simulink model "im_inv_model"  (R2026a)
settings: Solver=ode23tb  StopTime=param.sim.simlength  FixedStep=param.sim.tc  MaxStep=param.glb_time.tc  EnableMultiTasking=on
values from neighbouring files (symbols this model uses):
  param = struct()    [init_model.m]
undefined symbols (not defined in the file or in its folder): magnitude
libraries: fl_lib x53, nesl_utility x25, simulink x2, lithium_ion_battery x1, induction_machine x1, threephase_inductor_lib x1, dclink_with_center_tap x1, cstblocks_lti x1
(part 1 of 3)
settings Model: SimulationMode=accelerator  Creator=LTNBDA  LastModifiedBy=ltnbda
settings SolverCC: ZeroCrossControl=EnableAll
settings DataIOCC: MaxDataPoints=1  SignalLoggingSaveFormat=ModelDataLogs
settings OptimizationCC: InitFltsAndDblsToZero=on
settings DebuggingCC: SaveWithParameterizedLinksMsg=none  UnderspecifiedInitializationDetection=Classic  SignalResolutionControl=TryResolveAllWithWarning  MultiTaskDSMMsg=warning  MultiTaskCondExecSysMsg=none  MultiTaskRateTransMsg=warning
settings HardwareCC: ProdBitPerLong=64.0  ProdHWDeviceType=Generic->64-bit Embedded Processor (LP64)
settings SFSimCC: SimCustomHeaderCode=|
  | #include "mavgflt.h"
  | #include "mavgflt_simulink.h"
  | #include "bemf_obsv.h"
  | #include "bemf_obsv_simulink.h"
  | #include "bemf_obsv_load_est.h"
  | #include "bemf_obsv_load_est_simulink.h"
  | #include "dqvector_pi.h"
  | #include "dqvector_pi_simulink.h"
  | #include "sv_pwm_simulink.h"
  | #include "sv_pwm.h"
settings SFSimCC: SimUserSources=|
  | "mavgflt_simulink.c"
  | "mavgflt.c"
  | "bemf_obsv_simulink.c"
  | "bemf_obsv.c"
  | "bemf_obsv_load_est_simulink.c"
  | "bemf_obsv_load_est.c"
  | "dqvector_pi.c"
  | "dqvector_pi_simulink.c"
  | "sv_pwm_simulink.c"
  | "sv_pwm.c"
settings SFSimCC: SimUserIncludeDirs=|
  | include
  | src
settings GRTTargetCC: TargetFcnLib=ansi_tfl_tmw.mat  CombineOutputUpdateFcns=off  GRTInterface=on
settings SimscapeCC: SimscapeNormalizeSystem=off  SimscapeNominalValues="[{\"value\":\"1\",\"unit\":\"A\"},{\"value\":\"1\",\"unit\":\"bar\"},{\"value\":\"1\",\"unit\":\"cm^2\"},{\"value\":\"1\",\"unit\":\"cm^3/s\"},{\"value\":\"1\",\"unit\":\"kJ/kg\"},{\"value\":\"1\",\"unit\":\"kW\"},{\"value\":\"1\",\"unit\":\"l\"},{\"value\":\"1\",\"unit\":\"N\"},{\"value\":\"1\",\"unit\":\"N*m\"},{\"value\":\"1\",\"unit\":\"V\"}]"  SimscapeLogType=none  SimscapeLogDataHistory=5000.0

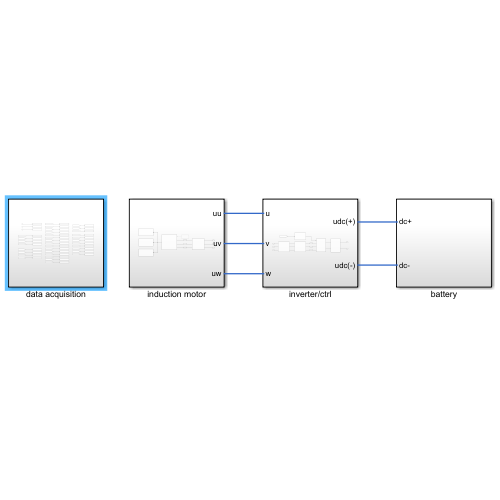
[thumbnail: Simulink's stored preview of the top-level diagram]
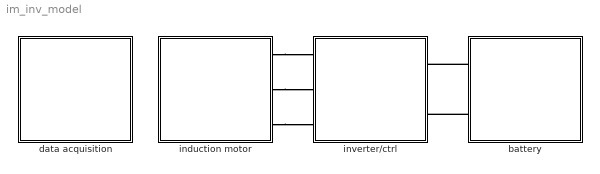
== system im_inv_model ==
  battery : Subsystem
  data acquisition : Subsystem
  induction motor : Subsystem
  inverter/ctrl : Subsystem
  connections:
  induction motor/RConn1 -- inverter/ctrl/LConn1
  induction motor/RConn2 -- inverter/ctrl/LConn2
  induction motor/RConn3 -- inverter/ctrl/LConn3
  battery/RConn1 -- inverter/ctrl/RConn1
  battery/RConn2 -- inverter/ctrl/RConn2

== system im_inv_model/battery ==
  To Workspace14 : ToWorkspace  VariableName=battery_data  SampleTime=param.glb_time.tc
      settings: MaxDataPoints=param.glb_time.Nc  Decimation=param.glb_time.decimation_tc
  lithium_ion_battery : lithium_ion_battery/lithium_ion_battery  Q=param.battery.pack_1.Q  number_of_cells=param.battery.pack_1.number_of_cells  E_1=param.battery.pack_1.E_1  E0=param.battery.pack_1.E0  E1=param.battery.pack_1.E1  E2=param.battery.pack_1.E2  E3=param.battery.pack_1.E3  Elog=param.battery.pack_1.Elog  R0=param.battery.pack_1.R0  R1=param.battery.pack_1.R1  C1=param.battery.pack_1.C1  M=param.battery.pack_1.M  alpha=param.battery.pack_1.alpha  soc_init=param.battery.pack_1.soc_init  ts_battery=param.glb_time.ts_dab  q1Kalman=param.battery.pack_1.q1Kalman  q2Kalman=param.battery.pack_1.q2Kalman  q3Kalman=param.battery.pack_1.q3Kalman  rKalman=param.battery.pack_1.rKalman  tc=param.glb_time.tc  enable_white_noise_m=0
  litium ion battery : Scope
      settings: ActiveDisplayYMinimum=-388.27149612119968  ActiveDisplayYMaximum=1221.0011073633038  DataLoggingVariableName=ScopeData3
  single_phase_ui_measure : Subsystem
  dc+ : PMIOPort  Side=Right
  dc- : PMIOPort  Port=2  Side=Right
  wires:
  lithium_ion_battery/1 -> To Workspace14/1, litium ion battery/1
  connections:
  lithium_ion_battery/RConn2 -- single_phase_ui_measure/LConn2
  single_phase_ui_measure/RConn1 -- dc+/RConn1
  lithium_ion_battery/RConn1 -- single_phase_ui_measure/LConn1
  dc-/RConn1 -- single_phase_ui_measure/RConn2

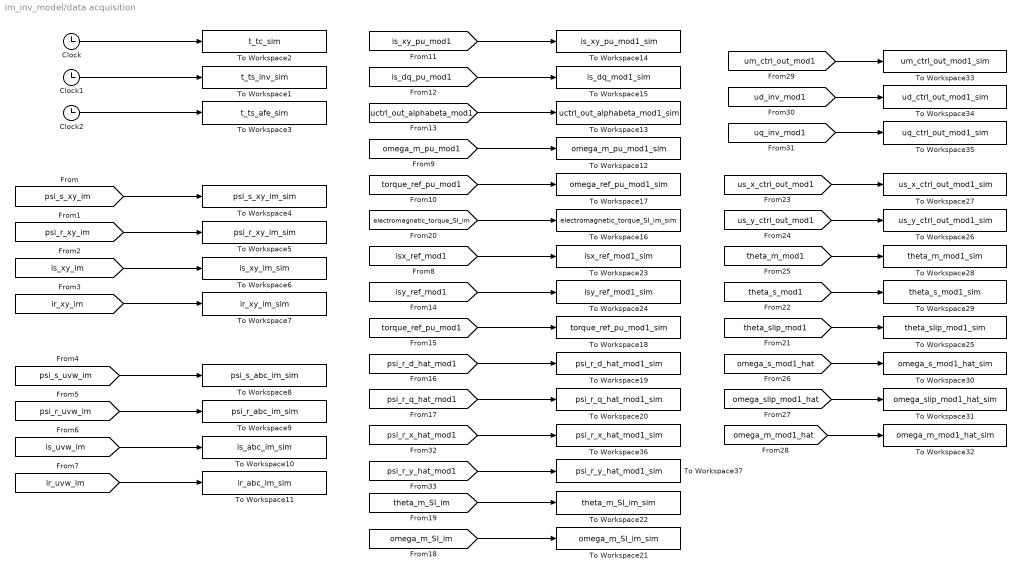
== system im_inv_model/data acquisition ==
  Clock : Clock
  Clock1 : Clock
  Clock2 : Clock
  To Workspace1 : ToWorkspace  VariableName=t_ts_inv_sim  SampleTime=param.glb_time.ts_inv
      settings: MaxDataPoints=param.glb_time.Ns_inv
  To Workspace10 : ToWorkspace  VariableName=is_abc_im_sim  SampleTime=param.glb_time.tc
      settings: MaxDataPoints=param.glb_time.Nc  Decimation=param.glb_time.decimation_tc
  To Workspace11 : ToWorkspace  VariableName=ir_abc_im_sim  SampleTime=param.glb_time.tc
      settings: MaxDataPoints=param.glb_time.Nc  Decimation=param.glb_time.decimation_tc
  To Workspace12 : ToWorkspace  VariableName=omega_m_pu_mod1_sim  SampleTime=param.glb_time.ts_inv
      settings: MaxDataPoints=param.glb_time.Ns_inv
  To Workspace13 : ToWorkspace  VariableName=uctrl_out_alphabeta_mod1_sim  SampleTime=param.glb_time.ts_inv
      settings: MaxDataPoints=param.glb_time.Ns_inv
  To Workspace14 : ToWorkspace  VariableName=is_xy_pu_mod1_sim  SampleTime=param.glb_time.ts_inv
      settings: MaxDataPoints=param.glb_time.Ns_inv
  To Workspace15 : ToWorkspace  VariableName=is_dq_mod1_sim  SampleTime=param.glb_time.ts_inv
      settings: MaxDataPoints=param.glb_time.Ns_inv
  To Workspace16 : ToWorkspace  VariableName=electromagnetic_torque_SI_im_sim  SampleTime=param.glb_time.ts_inv
      settings: MaxDataPoints=param.glb_time.Ns_inv
  To Workspace17 : ToWorkspace  VariableName=omega_ref_pu_mod1_sim  SampleTime=param.glb_time.ts_inv
      settings: MaxDataPoints=param.glb_time.Ns_inv
  To Workspace18 : ToWorkspace  VariableName=torque_ref_pu_mod1_sim  SampleTime=param.glb_time.ts_inv
      settings: MaxDataPoints=param.glb_time.Ns_inv
  To Workspace19 : ToWorkspace  VariableName=psi_r_d_hat_mod1_sim  SampleTime=param.glb_time.ts_inv
      settings: MaxDataPoints=param.glb_time.Ns_inv
  To Workspace2 : ToWorkspace  VariableName=t_tc_sim  SampleTime=param.glb_time.tc
      settings: MaxDataPoints=param.glb_time.Nc  Decimation=param.glb_time.decimation_tc
  To Workspace20 : ToWorkspace  VariableName=psi_r_q_hat_mod1_sim  SampleTime=param.glb_time.ts_inv
      settings: MaxDataPoints=param.glb_time.Ns_inv
  To Workspace21 : ToWorkspace  VariableName=omega_m_SI_im_sim  SampleTime=param.glb_time.ts_inv
      settings: MaxDataPoints=param.glb_time.Ns_inv
  To Workspace22 : ToWorkspace  VariableName=theta_m_SI_im_sim  SampleTime=param.glb_time.ts_inv
      settings: MaxDataPoints=param.glb_time.Ns_inv
  To Workspace23 : ToWorkspace  VariableName=isx_ref_mod1_sim  SampleTime=param.glb_time.ts_inv
      settings: MaxDataPoints=param.glb_time.Ns_inv
  To Workspace24 : ToWorkspace  VariableName=isy_ref_mod1_sim  SampleTime=param.glb_time.ts_inv
      settings: MaxDataPoints=param.glb_time.Ns_inv
  To Workspace25 : ToWorkspace  VariableName=theta_slip_mod1_sim  SampleTime=param.glb_time.ts_inv
      settings: MaxDataPoints=param.glb_time.Ns_inv
  To Workspace26 : ToWorkspace  VariableName=us_y_ctrl_out_mod1_sim  SampleTime=param.glb_time.ts_inv
      settings: MaxDataPoints=param.glb_time.Ns_inv
  To Workspace27 : ToWorkspace  VariableName=us_x_ctrl_out_mod1_sim  SampleTime=param.glb_time.ts_inv
      settings: MaxDataPoints=param.glb_time.Ns_inv
  To Workspace28 : ToWorkspace  VariableName=theta_m_mod1_sim  SampleTime=param.glb_time.ts_inv
      settings: MaxDataPoints=param.glb_time.Ns_inv
  To Workspace29 : ToWorkspace  VariableName=theta_s_mod1_sim  SampleTime=param.glb_time.ts_inv
      settings: MaxDataPoints=param.glb_time.Ns_inv
  To Workspace3 : ToWorkspace  VariableName=t_ts_afe_sim  SampleTime=param.glb_time.ts_inv
      settings: MaxDataPoints=param.glb_time.Ns_inv
  To Workspace30 : ToWorkspace  VariableName=omega_s_mod1_hat_sim  SampleTime=param.glb_time.ts_inv
      settings: MaxDataPoints=param.glb_time.Ns_inv
  To Workspace31 : ToWorkspace  VariableName=omega_slip_mod1_hat_sim  SampleTime=param.glb_time.ts_inv
      settings: MaxDataPoints=param.glb_time.Ns_inv
  To Workspace32 : ToWorkspace  VariableName=omega_m_mod1_hat_sim  SampleTime=param.glb_time.ts_inv
      settings: MaxDataPoints=param.glb_time.Ns_inv
  To Workspace33 : ToWorkspace  VariableName=um_ctrl_out_mod1_sim  SampleTime=param.glb_time.ts_inv
      settings: MaxDataPoints=param.glb_time.Ns_inv
  To Workspace34 : ToWorkspace  VariableName=ud_ctrl_out_mod1_sim  SampleTime=param.glb_time.ts_inv
      settings: MaxDataPoints=param.glb_time.Ns_inv
  To Workspace35 : ToWorkspace  VariableName=uq_ctrl_out_mod1_sim  SampleTime=param.glb_time.ts_inv
      settings: MaxDataPoints=param.glb_time.Ns_inv
  To Workspace36 : ToWorkspace  VariableName=psi_r_x_hat_mod1_sim  SampleTime=param.glb_time.ts_inv
      settings: MaxDataPoints=param.glb_time.Ns_inv
  To Workspace37 : ToWorkspace  VariableName=psi_r_y_hat_mod1_sim  SampleTime=param.glb_time.ts_inv
      settings: MaxDataPoints=param.glb_time.Ns_inv
  To Workspace4 : ToWorkspace  VariableName=psi_s_xy_im_sim  SampleTime=param.glb_time.tc
      settings: MaxDataPoints=param.glb_time.Nc  Decimation=param.glb_time.decimation_tc
  To Workspace5 : ToWorkspace  VariableName=psi_r_xy_im_sim  SampleTime=param.glb_time.tc
      settings: MaxDataPoints=param.glb_time.Nc  Decimation=param.glb_time.decimation_tc
  To Workspace6 : ToWorkspace  VariableName=is_xy_im_sim  SampleTime=param.glb_time.tc
      settings: MaxDataPoints=param.glb_time.Nc  Decimation=param.glb_time.decimation_tc
  To Workspace7 : ToWorkspace  VariableName=ir_xy_im_sim  SampleTime=param.glb_time.tc
      settings: MaxDataPoints=param.glb_time.Nc  Decimation=param.glb_time.decimation_tc
  To Workspace8 : ToWorkspace  VariableName=psi_s_abc_im_sim  SampleTime=param.glb_time.tc
      settings: MaxDataPoints=param.glb_time.Nc  Decimation=param.glb_time.decimation_tc
  To Workspace9 : ToWorkspace  VariableName=psi_r_abc_im_sim  SampleTime=param.glb_time.tc
      settings: MaxDataPoints=param.glb_time.Nc  Decimation=param.glb_time.decimation_tc
  wires:
  Clock/1 -> To Workspace2/1
  Clock1/1 -> To Workspace1/1
  Clock2/1 -> To Workspace3/1
  [psi_s_xy_im] -> To Workspace4/1
  [psi_r_xy_im] -> To Workspace5/1
  [is_xy_im] -> To Workspace6/1
  [ir_xy_im] -> To Workspace7/1
  [psi_s_uvw_im] -> To Workspace8/1
  [psi_r_uvw_im] -> To Workspace9/1
  [is_uvw_im] -> To Workspace10/1
  [ir_uvw_im] -> To Workspace11/1
  [is_dq_pu_mod1] -> To Workspace15/1
  [uctrl_out_alphabeta_mod1] -> To Workspace13/1
  [is_xy_pu_mod1] -> To Workspace14/1
  [omega_m_pu_mod1] -> To Workspace12/1
  [electromagnetic_torque_SI_im] -> To Workspace16/1
  [torque_ref_pu_mod1] -> To Workspace17/1
  [omega_m_SI_im] -> To Workspace21/1
  [torque_ref_pu_mod1] -> To Workspace18/1
  [psi_r_d_hat_mod1] -> To Workspace19/1
  [psi_r_q_hat_mod1] -> To Workspace20/1
  [theta_m_SI_im] -> To Workspace22/1
  [isx_ref_mod1] -> To Workspace23/1
  [isy_ref_mod1] -> To Workspace24/1
  [theta_slip_mod1] -> To Workspace25/1
  [us_x_ctrl_out_mod1] -> To Workspace27/1
  [us_y_ctrl_out_mod1] -> To Workspace26/1
  [theta_m_mod1] -> To Workspace28/1
  [theta_s_mod1] -> To Workspace29/1
  [omega_s_mod1_hat] -> To Workspace30/1
  [omega_slip_mod1_hat] -> To Workspace31/1
  [omega_m_mod1_hat] -> To Workspace32/1
  [um_ctrl_out_mod1] -> To Workspace33/1
  [ud_inv_mod1] -> To Workspace34/1
  [uq_inv_mod1] -> To Workspace35/1
  [psi_r_x_hat_mod1] -> To Workspace36/1
  [psi_r_y_hat_mod1] -> To Workspace37/1

== system im_inv_model/induction motor ==
  Inductor : fl_lib/Electrical/Electrical Elements/Inductor  l=1e-6 H  r=0 Ohm  g=1e-9 1/Ohm  i_specify=off  i_priority=None  i=0 A  i_nominal_specify=off  i_nominal_value=1  i_nominal_unit=A  v_specify=off  v_priority=None  v=0 V  v_nominal_specify=off  v_nominal_value=1  v_nominal_unit=V  i_L_specify=off  i_L_priority=High  i_L=0 A  i_L_nominal_specify=off  i_L_nominal_value=1  i_L_nominal_unit=A
  Inductor1 : fl_lib/Electrical/Electrical Elements/Inductor  l=1e-6 H  r=0 Ohm  g=1e-9 1/Ohm  i_specify=off  i_priority=None  i=0 A  i_nominal_specify=off  i_nominal_value=1  i_nominal_unit=A  v_specify=off  v_priority=None  v=0 V  v_nominal_specify=off  v_nominal_value=1  v_nominal_unit=V  i_L_specify=off  i_L_priority=High  i_L=0 A  i_L_nominal_specify=off  i_L_nominal_value=1  i_L_nominal_unit=A
  Inductor2 : fl_lib/Electrical/Electrical Elements/Inductor  l=1e-6 H  r=0 Ohm  g=1e-9 1/Ohm  i_specify=off  i_priority=None  i=0 A  i_nominal_specify=off  i_nominal_value=1  i_nominal_unit=A  v_specify=off  v_priority=None  v=0 V  v_nominal_specify=off  v_nominal_value=1  v_nominal_unit=V  i_L_specify=off  i_L_priority=High  i_L=0 A  i_L_nominal_specify=off  i_L_nominal_value=1  i_L_nominal_unit=A
  control performance evaluation : Subsystem
  induction motor : Subsystem
  load generator : Subsystem  Commented=on
  machine performance evaluation : Subsystem
  mechanical data : Subsystem
  threephase_vi_measures_stack : Subsystem
  uu : PMIOPort  Side=Right
  uv : PMIOPort  Port=2  Side=Right
  uw : PMIOPort  Port=3  Side=Right
  wires:
  induction motor/1(motor_data) -> control performance evaluation/1(machine_data), machine performance evaluation/1(machine_data), mechanical data/1(machine data)
  load generator/1(torque) -> induction motor/1(torque load)
  connections:
  induction motor/LConn2 -- Inductor1/LConn1
  threephase_vi_measures_stack/RConn1 -- Inductor/RConn1
  induction motor/LConn3 -- Inductor2/LConn1
  induction motor/LConn1 -- Inductor/LConn1
  threephase_vi_measures_stack/RConn2 -- Inductor1/RConn1
  threephase_vi_measures_stack/RConn3 -- Inductor2/RConn1
  threephase_vi_measures_stack/LConn1 -- uu/RConn1
  threephase_vi_measures_stack/LConn2 -- uv/RConn1
  threephase_vi_measures_stack/LConn3 -- uw/RConn1

== system im_inv_model/inverter//ctrl ==
  Inductor : fl_lib/Electrical/Electrical Elements/Inductor  l=1e-6 H  r=0 Ohm  g=1e-9 1/Ohm  i_specify=off  i_priority=None  i=0 A  i_nominal_specify=off  i_nominal_value=1  i_nominal_unit=A  v_specify=off  v_priority=None  v=0 V  v_nominal_specify=off  v_nominal_value=1  v_nominal_unit=V  i_L_specify=off  i_L_priority=High  i_L=0 A  i_L_nominal_specify=off  i_L_nominal_value=1  i_L_nominal_unit=A
  Inductor1 : fl_lib/Electrical/Electrical Elements/Inductor  l=1e-6 H  r=0 Ohm  g=1e-9 1/Ohm  i_specify=off  i_priority=None  i=0 A  i_nominal_specify=off  i_nominal_value=1  i_nominal_unit=A  v_specify=off  v_priority=None  v=0 V  v_nominal_specify=off  v_nominal_value=1  v_nominal_unit=V  i_L_specify=off  i_L_priority=High  i_L=0 A  i_L_nominal_specify=off  i_L_nominal_value=1  i_L_nominal_unit=A
  Inductor2 : fl_lib/Electrical/Electrical Elements/Inductor  l=1e-6 H  r=0 Ohm  g=1e-9 1/Ohm  i_specify=off  i_priority=None  i=0 A  i_nominal_specify=off  i_nominal_value=1  i_nominal_unit=A  v_specify=off  v_priority=None  v=0 V  v_nominal_specify=off  v_nominal_value=1  v_nominal_unit=V  i_L_specify=off  i_L_priority=High  i_L=0 A  i_L_nominal_specify=off  i_L_nominal_value=1  i_L_nominal_unit=A
  LFi : threephase_inductor_lib/threephase inductor  Lp=param.inv.hw.LFi H  L0=param.inv.hw.LFi_cm H  Rp=param.inv.hw.RLFi Ohm  R0=param.inv.hw.RLFi_cm Ohm  Lls=5e-6 H  uu_1_specify=off  uu_1_priority=None  uu_1=0 V  uu_1_nominal_specify=off  uu_1_nominal_value=1  uu_1_nominal_unit=V  uv_1_specify=off  uv_1_priority=None  uv_1=0 V  uv_1_nominal_specify=off  uv_1_nominal_value=1  uv_1_nominal_unit=V  uw_1_specify=off  uw_1_priority=None  uw_1=0 V  uw_1_nominal_specify=off  uw_1_nominal_value=1  uw_1_nominal_unit=V  uu_2_specify=off  uu_2_priority=None  uu_2=0 V  uu_2_nominal_specify=off  uu_2_nominal_value=1  uu_2_nominal_unit=V  uv_2_specify=off  uv_2_priority=None  uv_2=0 V  uv_2_nominal_specify=off  uv_2_nominal_value=1  uv_2_nominal_unit=V  uw_2_specify=off  uw_2_priority=None  uw_2=0 V  uw_2_nominal_specify=off  uw_2_nominal_value=1  uw_2_nominal_unit=V  iu_specify=off  iu_priority=None  iu=0 A  iu_nominal_specify=off  iu_nominal_value=1  iu_nominal_unit=A  iv_specify=off  iv_priority=None  iv=0 A  iv_nominal_specify=off  iv_nominal_value=1  iv_nominal_unit=A  iw_specify=off  iw_priority=None  iw=0 A  iw_nominal_specify=off  iw_nominal_value=1  iw_nominal_unit=A
  dc_source : Subsystem
  im_ctrl : Subsystem
  inverter : Subsystem
  threephase_vi_measures_stack : Subsystem
  u : PMIOPort  Side=Left
  v : PMIOPort  Port=2  Side=Left
  w : PMIOPort  Port=3  Side=Left
  udc(+) : PMIOPort  Port=4  Side=Right
  udc(-) : PMIOPort  Port=5  Side=Right
  wires:
  [theta_m_mod1] -> im_ctrl/1(theta_m)
  im_ctrl/1(u_ctrl_alphabeta) -> inverter/1(uab)
  connections:
  LFi/RConn1 -- Inductor/LConn1
  Inductor1/LConn1 -- LFi/RConn2
  LFi/RConn3 -- Inductor2/LConn1
  threephase_vi_measures_stack/LConn1 -- LFi/LConn1
  threephase_vi_measures_stack/LConn2 -- LFi/LConn2
  threephase_vi_measures_stack/LConn3 -- LFi/LConn3
  threephase_vi_measures_stack/RConn3 -- w/RConn1
  threephase_vi_measures_stack/RConn2 -- v/RConn1
  threephase_vi_measures_stack/RConn1 -- u/RConn1
  inverter/LConn1 -- Inductor/RConn1
  inverter/LConn2 -- Inductor1/RConn1
  inverter/LConn3 -- Inductor2/RConn1
  dc_source/RConn1 -- inverter/RConn1
  dc_source/RConn2 -- inverter/RConn2
  dc_source/LConn1 -- udc(+)/RConn1
  dc_source/LConn2 -- udc(-)/RConn1

== system im_inv_model/battery/single_phase_ui_measure ==
  Bus Creator : BusCreator  Inputs=2
  Current Sensor : fl_lib/Electrical/Electrical Sensors/Current Sensor
  Selector : Selector  InputPortWidth=2  IndexOptions=Index vector (dialog)  Indices=2  OutputSizes=1
  Selector1 : Selector  InputPortWidth=2  IndexOptions=Index vector (dialog)  Indices=1  OutputSizes=1
  Voltage Sensor : fl_lib/Electrical/Electrical Sensors/Voltage Sensor
  dab input modA : Scope  NumInputPorts=2
      settings: ActiveDisplayYMinimum=-2114.9540849373507  ActiveDisplayYMaximum=18648.004171529876  DataLoggingVariableName=ScopeData2
  iph : nesl_utility/PS-Simulink Converter  PhysicalDomain=network_engine_domain  SubClassName=ps_output  LeftPortType=input  RightPortType=output  PseudoPeriodic=off  Frequencies=[]  VectorFormat=1-D array  Unit=A  AffineConversion=off
  uph : nesl_utility/PS-Simulink Converter  PhysicalDomain=network_engine_domain  SubClassName=ps_output  LeftPortType=input  RightPortType=output  PseudoPeriodic=off  Frequencies=[]  VectorFormat=1-D array  Unit=V  AffineConversion=off
  Udc(+) : PMIOPort  Side=Left
  udc(+) : PMIOPort  Port=2  Side=Right
  Udc(-) : PMIOPort  Port=3  Side=Left
  udc(-) : PMIOPort  Port=4  Side=Right
  tag scope: current_battery=global, voltage_battery=global
  wires:
  Bus Creator/1 -> Selector/1, Selector1/1  "ui_data"
  iph/1 -> Bus Creator/1  "iph"
  uph/1 -> Bus Creator/2  "uph"
  Selector1/1 -> [current_battery], dab input modA/1  "current_battery"
  Selector/1 -> dab input modA/2, [voltage_battery]  "voltage_battery"
  connections:
  iph/LConn1 -- Current Sensor/RConn1
  Voltage Sensor/LConn1 -- Current Sensor/LConn1 -- Udc(+)/RConn1
  Current Sensor/RConn2 -- udc(+)/RConn1
  Voltage Sensor/RConn1 -- uph/LConn1
  Voltage Sensor/RConn2 -- Udc(-)/RConn1 -- udc(-)/RConn1

== system im_inv_model/induction motor/control performance evaluation ==
  machine_data : Inport
  adc2dq_s_1 : Subsystem
  adc2dq_s_2 : Subsystem
  adc2dq_slip_1 : Subsystem
  adc2dq_slip_2 : Subsystem
  ir_uvw : BusSelector  OutputSignals=iru(A),irv(A),irw(A)  OutputAsBus=on
  is_uvw : BusSelector  OutputSignals=isu(A),isv(A),isw(A)  OutputAsBus=on
  psi_r_uvw : BusSelector  OutputSignals=psi_r_u(Vs),psi_r_v(Vs),psi_r_w(Vs)  OutputAsBus=on
  psi_s_uvw : BusSelector  OutputSignals=psi_s_u(Vs),psi_s_v(Vs),psi_s_w(Vs)  OutputAsBus=on
  stator/rotor uvw currents : Scope  NumInputPorts=2
      settings: ActiveDisplayYMinimum=-767.52442584692187  ActiveDisplayYMaximum=813.0675363801156  DataLoggingVariableName=ScopeData15
  stator/rotor uvw fluxes : Scope  NumInputPorts=2
      settings: ActiveDisplayYMinimum=-1.236467692960036  ActiveDisplayYMaximum=1.3517472693614645  DataLoggingVariableName=ScopeData16
  stator/rotor xy currents : Scope  NumInputPorts=2
      settings: ActiveDisplayYMinimum=-2297.8110392737149  ActiveDisplayYMaximum=257.87338844640192
  stator/rotor xy fluxes : Scope  NumInputPorts=2
      settings: ActiveDisplayYMinimum=-2.073456127351001  ActiveDisplayYMaximum=0.70751576648044434  DataLoggingVariableName=ScopeData2
  tag scope: ir_uvw_im=global, is_uvw_im=global, psi_r_uvw_im=global, psi_s_uvw_im=global
  wires:
  machine_data/1 -> psi_s_uvw/1, psi_r_uvw/1, is_uvw/1, ir_uvw/1
  psi_s_uvw/1 -> [psi_s_uvw_im], adc2dq_s_1/1(abc)
  adc2dq_s_1/1(dq) -> stator/rotor xy fluxes/1  "psi_s_xy"
  psi_r_uvw/1 -> [psi_r_uvw_im], adc2dq_slip_1/1(abc)
  adc2dq_slip_1/1(dq) -> stator/rotor xy fluxes/2  "psi_r_xy"
  adc2dq_slip_2/1(dq) -> stator/rotor xy currents/2  "ir_xy"
  adc2dq_s_2/1(dq) -> stator/rotor xy currents/1  "is_xy"
  is_uvw/1 -> [is_uvw_im], adc2dq_s_2/1(abc)
  ir_uvw/1 -> [ir_uvw_im], adc2dq_slip_2/1(abc)
  [is_uvw_im] -> stator/rotor uvw currents/1
  [ir_uvw_im] -> stator/rotor uvw currents/2
  [psi_r_uvw_im] -> stator/rotor uvw fluxes/2
  [psi_s_uvw_im] -> stator/rotor uvw fluxes/1

== system im_inv_model/induction motor/induction motor ==
  torque load : Inport
  Gain : Gain  Gain=-1
  Ideal Rotational Motion Sensor : fl_lib/Mechanical/Mechanical Sensors/Ideal Rotational Motion Sensor  reference=foundation.enum.MeasurementReference.difference  acceleration_port=false  velocity_port=true  position_port=true  wrap_angle=false  offset=0 rad
  Ideal Torque Source : fl_lib/Mechanical/Mechanical Sources/Ideal Torque Source
  Mechanical Rotational Reference : fl_lib/Mechanical/Rotational Elements/Mechanical Rotational Reference
  Mechanical Rotational Reference1 : fl_lib/Mechanical/Rotational Elements/Mechanical Rotational Reference
  Open Circuit : fl_lib/Electrical/Electrical Elements/Open Circuit  v_specify=off  v_priority=None  v=0 V  v_nominal_specify=off  v_nominal_value=1  v_nominal_unit=V
  PS Gain : fl_lib/Physical Signals/Functions/PS Gain  gain=-1
  PS Transfer Function : fl_lib/Physical Signals/Linear Operators/PS Transfer Function  transfer_function_type=foundation.enum.transfer_function_type.lag  T=1/50 s  T1=2 s  T2=1 s  reset_method=foundation.enum.IntegratorResetSpec.None  initial_condition_spec=foundation.enum.IntegratorICSpec.Internal  y0=0 N*m
  PS-Simulink Converter24 : nesl_utility/PS-Simulink Converter  PhysicalDomain=network_engine_domain  SubClassName=ps_output  LeftPortType=input  RightPortType=output  PseudoPeriodic=off  Frequencies=[]  VectorFormat=1-D array  Unit=rad  AffineConversion=off
  Simulink-PS Converter : nesl_utility/Simulink-PS Converter  PhysicalDomain=network_engine_domain  SubClassName=ps_input  LeftPortType=input  RightPortType=output  PseudoPeriodic=off  Frequencies=[]  NoiseDistribution=none  NoiseParameters=[]  Unit=N*m  AffineConversion=off  FilteringAndDerivatives=provide  SimscapeFilterOrder=1  InputFilterTimeConstant=0.001  UdotUserProvided=0
  poliphase_induction_machine1 : induction_machine/poliphase_induction_machine  Rs_m=param.im.machine.Rs  Ls_m=param.im.machine.Ls  Lm_m=param.im.machine.Lm  Lr_m=param.im.machine.Lr  Rr_m=param.im.machine.Rr  Jm_m=param.im.machine.Jm  bm_m=param.im.machine.load_friction  cp_m=param.im.machine.pp
  uu : PMIOPort  Side=Left
  uv : PMIOPort  Port=2  Side=Left
  uw : PMIOPort  Port=3  Side=Left
  motor_data : Outport
  tag scope: rotor_phase_m_encoder=global
  wires:
  torque load/1 -> Simulink-PS Converter/1
  PS-Simulink Converter24/1 -> Gain/1
  Gain/1 -> [rotor_phase_m_encoder]
  poliphase_induction_machine1/1 -> motor_data/1
  connections:
  Ideal Torque Source/LConn1 -- poliphase_induction_machine1/RConn1 -- Ideal Rotational Motion Sensor/RConn1
  Mechanical Rotational Reference/LConn1 -- Ideal Torque Source/RConn2
  PS Transfer Function/RConn1 -- PS Gain/LConn1
  Simulink-PS Converter/RConn1 -- PS Transfer Function/LConn1
  PS Gain/RConn1 -- Ideal Torque Source/RConn1
  Mechanical Rotational Reference1/LConn1 -- Ideal Rotational Motion Sensor/LConn1
  Ideal Rotational Motion Sensor/RConn3 -- PS-Simulink Converter24/LConn1
  poliphase_induction_machine1/LConn1 -- uu/RConn1
  poliphase_induction_machine1/LConn2 -- uv/RConn1
  poliphase_induction_machine1/LConn3 -- uw/RConn1
  Open Circuit/LConn1 -- poliphase_induction_machine1/LConn4

== system im_inv_model/induction motor/load generator ==
  Gain3 : Gain
  RampSlow : simulink/Sources/Ramp  slope=param.im.load.Tload/param.im.load.timeRamp/param.sim.simlength*2  start=param.im.load.start_load_ramp  InitialOutput=0
  Saturation : Saturate  UpperLimit=param.im.load.Tload  LowerLimit=-param.im.load.Tload
  Step : Step  FinalValue=param.im.load.Tload  SampleTime=0
  torque : Outport
  wires:
  Gain3/1 -> torque/1
  RampSlow/1 -> Saturation/1
  Step/1 -> Gain3/1

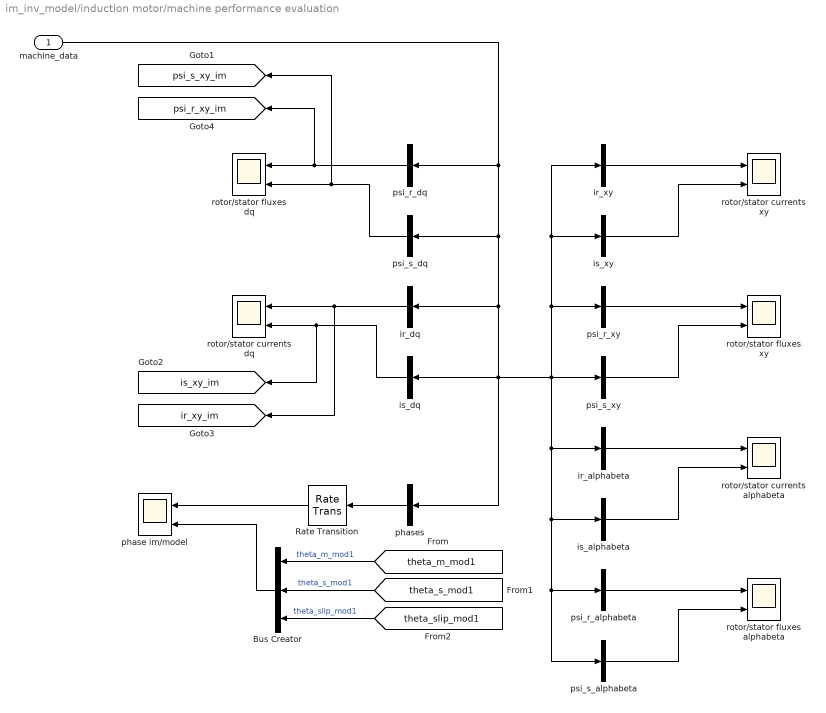
== system im_inv_model/induction motor/machine performance evaluation ==
  machine_data : Inport
  Bus Creator : BusCreator  Inputs=3
  Rate Transition : RateTransition
  ir_alphabeta : BusSelector  OutputSignals=ir_alpha(A),ir_beta(A)  OutputAsBus=on
  ir_dq : BusSelector  OutputSignals=ird(A),irq(A)  OutputAsBus=on
  ir_xy : BusSelector  OutputSignals=irx(A),iry(A)  OutputAsBus=on
  is_alphabeta : BusSelector  OutputSignals=is_alpha(A),is_beta(A)  OutputAsBus=on
  is_dq : BusSelector  OutputSignals="isd  (A),isq(A)"  OutputAsBus=on
  is_xy : BusSelector  OutputSignals=isx(A),isy(A)  OutputAsBus=on
  phase im/model : Scope  NumInputPorts=2
      settings: ActiveDisplayYMinimum=-3.9265862737533843  ActiveDisplayYMaximum=3.9260094563988228  DataLoggingVariableName=ScopeData17
  phases : BusSelector  OutputSignals=rotor_phase_electrical(rad),stator_phase_electrical(rad),slip_phase_electrical(rad)  OutputAsBus=on
  psi_r_alphabeta : BusSelector  OutputSignals=psi_r_alpha(Vs),psi_r_beta(Vs)  OutputAsBus=on
  psi_r_dq : BusSelector  OutputSignals=psi_r_d(Vs),psi_r_q(Vs)  OutputAsBus=on
  psi_r_xy : BusSelector  OutputSignals=psi_r_x(Vs),psi_r_y(Vs)  OutputAsBus=on
  psi_s_alphabeta : BusSelector  OutputSignals=psi_s_alpha(Vs),psi_s_beta(Vs)  OutputAsBus=on
  psi_s_dq : BusSelector  OutputSignals=psi_s_d(Vs),psi_s_q(Vs)  OutputAsBus=on
  psi_s_xy : BusSelector  OutputSignals=psi_s_x(Vs),psi_s_y(Vs)  OutputAsBus=on
  rotor/stator currents alphabeta : Scope  NumInputPorts=2
      settings: ActiveDisplayYMinimum=-755.39541757603456  ActiveDisplayYMaximum=755.78854721223524  DataLoggingVariableName=ScopeData13
  rotor/stator currents dq : Scope  NumInputPorts=2
      settings: ActiveDisplayYMinimum=-890.18338057152221  ActiveDisplayYMaximum=1029.0815378849704  DataLoggingVariableName=ScopeData3
  rotor/stator currents xy : Scope  NumInputPorts=2
      settings: ActiveDisplayYMinimum=-752.721270314659  ActiveDisplayYMaximum=755.87183047398014  DataLoggingVariableName=ScopeData6
  rotor/stator fluxes alphabeta : Scope  NumInputPorts=2
      settings: ActiveDisplayYMinimum=-2.3042822009960924  ActiveDisplayYMaximum=2.3048133761652672  DataLoggingVariableName=ScopeData14
  rotor/stator fluxes dq : Scope  NumInputPorts=2
      settings: ActiveDisplayYMinimum=-1.3704704510731207  ActiveDisplayYMaximum=1.3704905297766097
  rotor/stator fluxes xy : Scope  NumInputPorts=2
      settings: ActiveDisplayYMinimum=-1.4064321862490787  ActiveDisplayYMaximum=1.4064895725533888  DataLoggingVariableName=ScopeData12
  tag scope: ir_xy_im=global, is_xy_im=global, psi_r_xy_im=global, psi_s_xy_im=global
  wires:
  psi_r_dq/1 -> [psi_r_xy_im], rotor/stator fluxes dq/1
  psi_s_dq/1 -> [psi_s_xy_im], rotor/stator fluxes dq/2
  ir_dq/1 -> [ir_xy_im], rotor/stator currents dq/1
  is_dq/1 -> [is_xy_im], rotor/stator currents dq/2
  is_xy/1 -> rotor/stator currents xy/2
  ir_xy/1 -> rotor/stator currents xy/1
  psi_r_xy/1 -> rotor/stator fluxes xy/1
  psi_s_xy/1 -> rotor/stator fluxes xy/2
  psi_s_alphabeta/1 -> rotor/stator fluxes alphabeta/2
  psi_r_alphabeta/1 -> rotor/stator fluxes alphabeta/1
  machine_data/1 -> psi_r_dq/1, ir_dq/1, phases/1, psi_s_alphabeta/1, psi_r_alphabeta/1, is_alphabeta/1, ir_alphabeta/1, psi_s_xy/1, ir_xy/1, is_xy/1, psi_r_xy/1, is_dq/1, psi_s_dq/1
  ir_alphabeta/1 -> rotor/stator currents alphabeta/1
  is_alphabeta/1 -> rotor/stator currents alphabeta/2
  phases/1 -> Rate Transition/1
  [theta_m_mod1] -> Bus Creator/1  "theta_m_mod1"
  [theta_slip_mod1] -> Bus Creator/3  "theta_slip_mod1"
  Bus Creator/1 -> phase im/model/2
  [theta_s_mod1] -> Bus Creator/2  "theta_s_mod1"
  Rate Transition/1 -> phase im/model/1

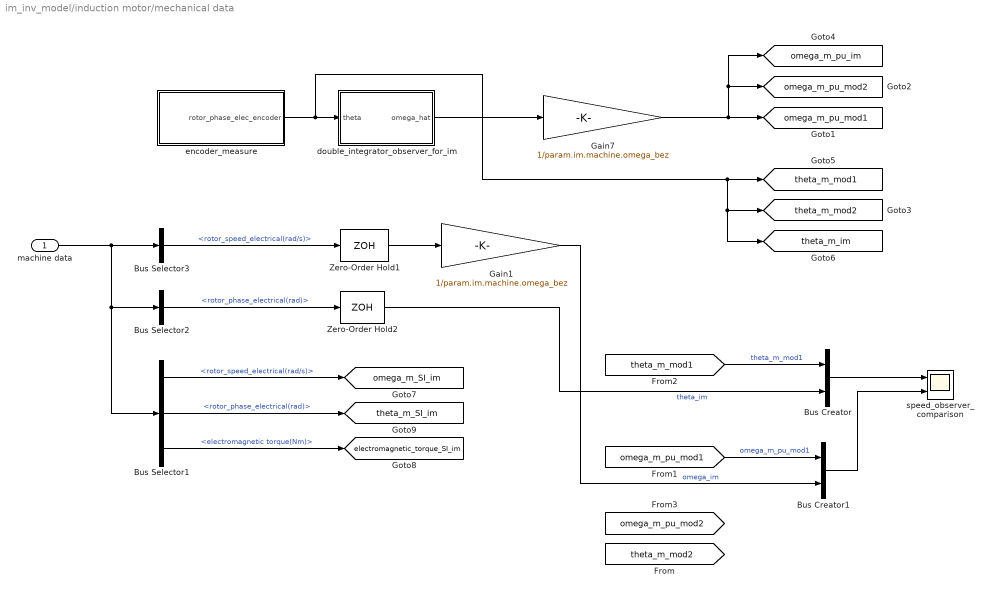
== system im_inv_model/induction motor/mechanical data ==
  machine data : Inport
  Bus Creator : BusCreator  Inputs=2
  Bus Creator1 : BusCreator  Inputs=2
  Bus Selector1 : BusSelector  OutputSignals=rotor_speed_electrical(rad/s),rotor_phase_electrical(rad),electromagnetic torque(Nm)
  Bus Selector2 : BusSelector  OutputSignals=rotor_phase_electrical(rad)
  Bus Selector3 : BusSelector  OutputSignals=rotor_speed_electrical(rad/s)
  Gain1 : Gain  Gain=1/param.im.machine.omega_bez
  Gain7 : Gain  Gain=1/param.im.machine.omega_bez
  Zero-Order Hold1 : ZeroOrderHold  SampleTime=param.glb_time.ts_inv
  Zero-Order Hold2 : ZeroOrderHold  SampleTime=param.glb_time.ts_inv
  double_integrator_observer_for_im : Subsystem
  encoder_measure : Subsystem
  speed_observer_comparison : Scope  NumInputPorts=2
      settings: ActiveDisplayYMinimum=-0.069232829506416654  ActiveDisplayYMaximum=0.62309538771470585  DataLoggingVariableName=ScopeData8
  tag scope: electromagnetic_torque_SI_im=global, omega_m_SI_im=global, omega_m_pu_im=global, omega_m_pu_mod1=global, omega_m_pu_mod2=global, theta_m_SI_im=global, theta_m_im=global, theta_m_mod1=global, theta_m_mod2=global
  wires:
  encoder_measure/1(rotor_phase_elec_encoder) -> [theta_m_mod1], [theta_m_im], [theta_m_mod2], double_integrator_observer_for_im/1(theta)
  machine data/1 -> Bus Selector1/1, Bus Selector2/1, Bus Selector3/1
  Bus Selector3/1 -> Zero-Order Hold1/1  "<rotor_speed_electrical(rad/s)>"
  Bus Selector2/1 -> Zero-Order Hold2/1  "<rotor_phase_electrical(rad)>"
  Gain7/1 -> [omega_m_pu_mod1], [omega_m_pu_mod2], [omega_m_pu_im]
  Bus Selector1/1 -> [omega_m_SI_im]  "<rotor_speed_electrical(rad/s)>"
  Bus Selector1/3 -> [electromagnetic_torque_SI_im]  "<electromagnetic torque(Nm)>"
  Bus Selector1/2 -> [theta_m_SI_im]  "<rotor_phase_electrical(rad)>"
  double_integrator_observer_for_im/1(omega_hat) -> Gain7/1
  [theta_m_mod1] -> Bus Creator/1  "theta_m_mod1"
  [omega_m_pu_mod1] -> Bus Creator1/1  "omega_m_pu_mod1"
  Bus Creator/1 -> speed_observer_comparison/1
  Bus Creator1/1 -> speed_observer_comparison/2
  Zero-Order Hold2/1 -> Bus Creator/2  "theta_im"
  Zero-Order Hold1/1 -> Gain1/1
  Gain1/1 -> Bus Creator1/2  "omega_im"

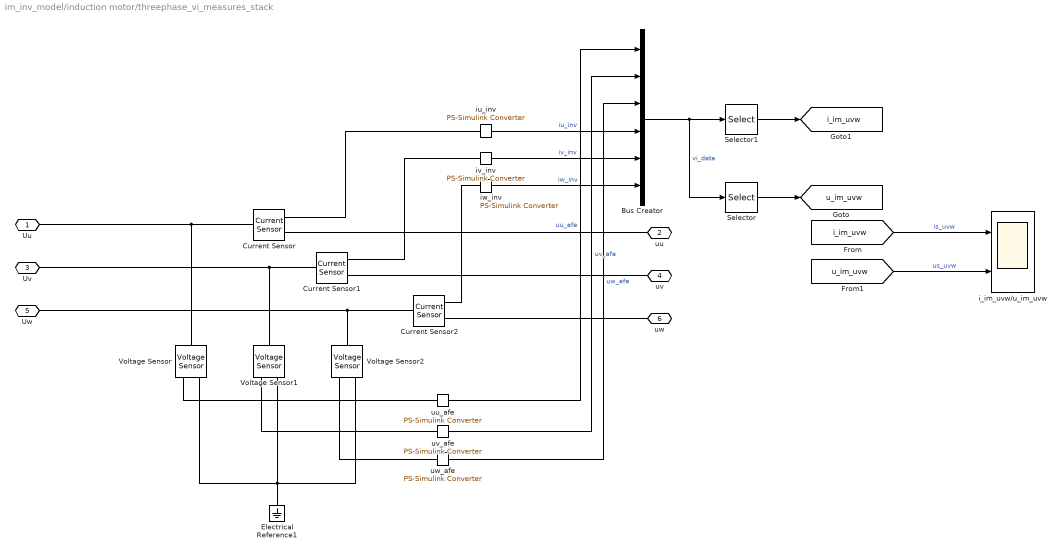
== system im_inv_model/induction motor/threephase_vi_measures_stack ==
  Bus Creator : BusCreator  Inputs=6
  Current Sensor : fl_lib/Electrical/Electrical Sensors/Current Sensor
  Current Sensor1 : fl_lib/Electrical/Electrical Sensors/Current Sensor
  Current Sensor2 : fl_lib/Electrical/Electrical Sensors/Current Sensor
  Electrical Reference1 : fl_lib/Electrical/Electrical Elements/Electrical Reference
  Selector : Selector  InputPortWidth=6  IndexOptions=Index vector (dialog)  Indices=[1 2 3]  OutputSizes=1
  Selector1 : Selector  InputPortWidth=6  IndexOptions=Index vector (dialog)  Indices=[4 5 6]  OutputSizes=1
  Voltage Sensor : fl_lib/Electrical/Electrical Sensors/Voltage Sensor
  Voltage Sensor1 : fl_lib/Electrical/Electrical Sensors/Voltage Sensor
  Voltage Sensor2 : fl_lib/Electrical/Electrical Sensors/Voltage Sensor
  i_im_uvw/u_im_uvw : Scope  NumInputPorts=2
      settings: ActiveDisplayYMinimum=-673.15802001560257  ActiveDisplayYMaximum=673.14084911315229
  iu_inv : nesl_utility/PS-Simulink Converter  PhysicalDomain=network_engine_domain  SubClassName=ps_output  LeftPortType=input  RightPortType=output  PseudoPeriodic=off  Frequencies=[]  VectorFormat=1-D array  Unit=A  AffineConversion=off
  iv_inv : nesl_utility/PS-Simulink Converter  PhysicalDomain=network_engine_domain  SubClassName=ps_output  LeftPortType=input  RightPortType=output  PseudoPeriodic=off  Frequencies=[]  VectorFormat=1-D array  Unit=A  AffineConversion=off
  iw_inv : nesl_utility/PS-Simulink Converter  PhysicalDomain=network_engine_domain  SubClassName=ps_output  LeftPortType=input  RightPortType=output  PseudoPeriodic=off  Frequencies=[]  VectorFormat=1-D array  Unit=A  AffineConversion=off
  uu_afe : nesl_utility/PS-Simulink Converter  PhysicalDomain=network_engine_domain  SubClassName=ps_output  LeftPortType=input  RightPortType=output  PseudoPeriodic=off  Frequencies=[]  VectorFormat=1-D array  Unit=V  AffineConversion=off
  uv_afe : nesl_utility/PS-Simulink Converter  PhysicalDomain=network_engine_domain  SubClassName=ps_output  LeftPortType=input  RightPortType=output  PseudoPeriodic=off  Frequencies=[]  VectorFormat=1-D array  Unit=V  AffineConversion=off
  uw_afe : nesl_utility/PS-Simulink Converter  PhysicalDomain=network_engine_domain  SubClassName=ps_output  LeftPortType=input  RightPortType=output  PseudoPeriodic=off  Frequencies=[]  VectorFormat=1-D array  Unit=V  AffineConversion=off
  Uu : PMIOPort  Side=Left
  uu : PMIOPort  Port=2  Side=Right
  Uv : PMIOPort  Port=3  Side=Left
  uv : PMIOPort  Port=4  Side=Right
  Uw : PMIOPort  Port=5  Side=Left
  uw : PMIOPort  Port=6  Side=Right
  tag scope: i_im_uvw=global, u_im_uvw=global
  wires:
  Bus Creator/1 -> Selector1/1, Selector/1  "vi_data"
  Selector/1 -> [u_im_uvw]
  iv_inv/1 -> Bus Creator/5  "iv_inv"
  iu_inv/1 -> Bus Creator/4  "iu_inv"
  iw_inv/1 -> Bus Creator/6  "iw_inv"
  uu_afe/1 -> Bus Creator/1  "uu_afe"
  uv_afe/1 -> Bus Creator/2  "uv_afe"
  uw_afe/1 -> Bus Creator/3  "uw_afe"
  Selector1/1 -> [i_im_uvw]
  [i_im_uvw] -> i_im_uvw/u_im_uvw/1  "is_uvw"
  [u_im_uvw] -> i_im_uvw/u_im_uvw/2  "us_uvw"
  connections:
  Current Sensor1/LConn1 -- Uv/RConn1 -- Voltage Sensor1/LConn1
  Electrical Reference1/LConn1 -- Voltage Sensor/RConn2 -- Voltage Sensor2/RConn2 -- Voltage Sensor1/RConn2
  Voltage Sensor/RConn1 -- uu_afe/LConn1
  Current Sensor/RConn2 -- uu/RConn1
  Voltage Sensor1/RConn1 -- uv_afe/LConn1
  Voltage Sensor2/LConn1 -- Uw/RConn1 -- Current Sensor2/LConn1
  Current Sensor/LConn1 -- Uu/RConn1 -- Voltage Sensor/LConn1
  Current Sensor1/RConn2 -- uv/RConn1
  Voltage Sensor2/RConn1 -- uw_afe/LConn1
  iv_inv/LConn1 -- Current Sensor1/RConn1
  iu_inv/LConn1 -- Current Sensor/RConn1
  iw_inv/LConn1 -- Current Sensor2/RConn1
  Current Sensor2/RConn2 -- uw/RConn1

== system im_inv_model/inverter//ctrl/dc_source ==
  Bus Selector : BusSelector  OutputSignals=udc,Cdc1_current,vdc_pu
  Electrical Reference : fl_lib/Electrical/Electrical Elements/Electrical Reference
  Solver Configuration : nesl_utility/Solver Configuration  PhysicalDomain=network_engine_domain  SubClassName=solver  LeftPortType=input  RightPortType=generic  Tones=[]  Harmonics=[]  SimulateNoise=off  Profile=off  UseLocalSampling=off  EnableSwitchedLinearOptims=on  FrequencyDomain=off  UseCCode=off  RelTol=0.001  AbsTol=0.001  MinStep=1e-09  ToWorkspace=off  RevertToSquareIcSolve=off  NumHomotopyIterations=100  PhasorMode=off  PhasorModeNumHarmonics=1  ConsistencySolver=NEWTON_XTOL_AFTER_FTOL  CanonicalOrdering=UNORDERED  OptimizeIntermediates=UNOPTIMIZED  IndexReductionMethod=DerivativeReplacement  DoDC=on  ResidualTolerance=1e-09  ConsistencyTolSource=GLOBAL  ConsistencyAbsTol=0.001  ConsistencyRelTol=0.001  ConsistencyTolFactor=0.001  UseLocalSolver=on  LocalSolverChoice=NE_BACKWARD_EULER_ADVANCER  ResolveIndetEquations=on  FunctionEvalNumThread=1  LocalSolverSampleTime=param.glb_time.tc  DoFixedCost=on  MaxNonlinIter=param.sim.nonlinear_iterations  MaxModeIter=2  ComputeImpulses=off  ImpulseIterations=2  LinearAlgebra=auto  LinearAlgebraNumThread=0  EquationFormulation=NE_TIME_EF  DelaysMemoryBudget=1024  AutomaticFiltering=on  FilteringTimeConstant=0.001  PartitionStorageMethod=AS_NEEDED  PartitionMemoryBudget=1024  PartitionMethod=ROBUST  MultibodyUseLocalSolver=off  MultibodyLocalSolverChoice=ODE1  MultibodyLocalSolverSampleTime=0.001
  dclink : dclink_with_center_tap/dclink  Cdc1=param.inv.hw.CFi1  Cdc2=param.inv.hw.CFi2  Rudc_measure=param.inv.hw.Rudc_measure  Vdc_scale=param.inv.hw.udc_nom
  udc(+) : PMIOPort  Side=Right
  udc(-) : PMIOPort  Port=2  Side=Right
  Udc(+) : PMIOPort  Port=3  Side=Left
  Udc(-) : PMIOPort  Port=4  Side=Left
  tag scope: all_voltages_about_dclink=global, ic_dclink_mod1=global, udc_mod1=global, vdc_pu_inv_mod1=global
  wires:
  dclink/1 -> Bus Selector/1, [all_voltages_about_dclink]
  Bus Selector/1 -> [udc_mod1]  "<udc>"
  Bus Selector/2 -> [ic_dclink_mod1]  "<Cdc1_current>"
  Bus Selector/3 -> [vdc_pu_inv_mod1]  "<vdc_pu>"
  connections:
  dclink/LConn1 -- udc(+)/RConn1
  Electrical Reference/LConn1 -- Solver Configuration/RConn1 -- dclink/RConn2
  udc(-)/RConn1 -- dclink/LConn2
  dclink/RConn3 -- Udc(-)/RConn1
  dclink/RConn1 -- Udc(+)/RConn1

== system im_inv_model/inverter//ctrl/im_ctrl ==
  theta_m : Inport
  Bus Creator : BusCreator  Inputs=3
  Mux : Mux  Inputs=2
  Mux1 : Mux  Inputs=2
  Mux2 : Mux  Inputs=2
  abc2dq : Subsystem
  "abc2dq " : Subsystem
  acquisition : Subsystem
  dq2alphabeta : Subsystem
  im_control : Subsystem
  is_xy/umot : Scope  NumInputPorts=2
      settings: ActiveDisplayYMinimum=-0.99102773322183157  ActiveDisplayYMaximum=1.130445984899523  DataLoggingVariableName=ScopeData11
  u_ctrl_alphabeta : Outport  VectorParamsAs1DForOutWhenUnconnected=off
  tag scope: is_dq_pu_mod1=global, is_xy_pu_mod1=global, uctrl_out_alphabeta_mod1=global
  wires:
  Mux/1 -> [uctrl_out_alphabeta_mod1], u_ctrl_alphabeta/1
  Mux1/1 -> [is_xy_pu_mod1]
  im_control/1(usx) -> dq2alphabeta/1(x)
  im_control/2(usy) -> dq2alphabeta/2(y)
  dq2alphabeta/1(uctrl_alpha) -> Mux/1
  dq2alphabeta/2(uctrl_beta) -> Mux/2
  Mux2/1 -> [is_dq_pu_mod1]
  "abc2dq "/2(q) -> Mux2/2
  "abc2dq "/1(d) -> Mux2/1
  abc2dq/1(d) -> Mux1/1
  abc2dq/2(q) -> Mux1/2
  acquisition/2(iv) -> abc2dq/2(b), "abc2dq "/2(b)
  acquisition/1(iu) -> abc2dq/1(a), "abc2dq "/1(a)
  acquisition/3(iw) -> abc2dq/3(c), "abc2dq "/3(c)
  theta_m/1 -> "abc2dq "/4(wt)
  [theta_s_mod1] -> abc2dq/4(wt)
  im_control/3(theta_s) -> dq2alphabeta/3(theta_s)
  [is_xy_pu_mod1] -> is_xy/umot/1  "is_xy_pu_mod1"
  [ud_inv_mod1] -> Bus Creator/2  "ud"
  [um_ctrl_out_mod1] -> Bus Creator/1  "umot"
  [uq_inv_mod1] -> Bus Creator/3  "uq"
  Bus Creator/1 -> is_xy/umot/2

== system im_inv_model/inverter//ctrl/inverter ==
  uab : Inport
  Current Sensor : fl_lib/Electrical/Electrical Sensors/Current Sensor
  PS-Simulink Converter1 : nesl_utility/PS-Simulink Converter  PhysicalDomain=network_engine_domain  SubClassName=ps_output  LeftPortType=input  RightPortType=output  PseudoPeriodic=off  Frequencies=[]  VectorFormat=1-D array  Unit=A  AffineConversion=on
  PS-Simulink Converter4 : nesl_utility/PS-Simulink Converter  PhysicalDomain=network_engine_domain  SubClassName=ps_output  LeftPortType=input  RightPortType=output  PseudoPeriodic=off  Frequencies=[]  VectorFormat=1-D array  Unit=V  AffineConversion=on
  Transfer Fcn : TransferFcn  Denominator=[1e-2 1]
  Voltage Sensor : fl_lib/Electrical/Electrical Sensors/Voltage Sensor
  idc/udc : Scope  NumInputPorts=2
      settings: ActiveDisplayYMinimum=-13.479588708590834  ActiveDisplayYMaximum=121.31629837731754
  inverter : Subsystem
  Udc(+) : PMIOPort  Side=Right
  Udc(-) : PMIOPort  Port=2  Side=Right
  us_u : PMIOPort  Port=3  Side=Left
  us_v : PMIOPort  Port=4  Side=Left
  us_w : PMIOPort  Port=5  Side=Left
  wires:
  uab/1 -> inverter/1(uab)
  Transfer Fcn/1 -> idc/udc/1  "idc_flt"
  PS-Simulink Converter1/1 -> Transfer Fcn/1  "idc"
  PS-Simulink Converter4/1 -> idc/udc/2  "udc"
  connections:
  PS-Simulink Converter1/LConn1 -- Current Sensor/RConn1
  Current Sensor/RConn2 -- inverter/RConn1 -- Voltage Sensor/LConn1
  Current Sensor/LConn1 -- Udc(+)/RConn1
  Udc(-)/RConn1 -- inverter/RConn2 -- Voltage Sensor/RConn2
  us_w/RConn1 -- inverter/LConn3
  us_v/RConn1 -- inverter/LConn2
  us_u/RConn1 -- inverter/LConn1
  PS-Simulink Converter4/LConn1 -- Voltage Sensor/RConn1

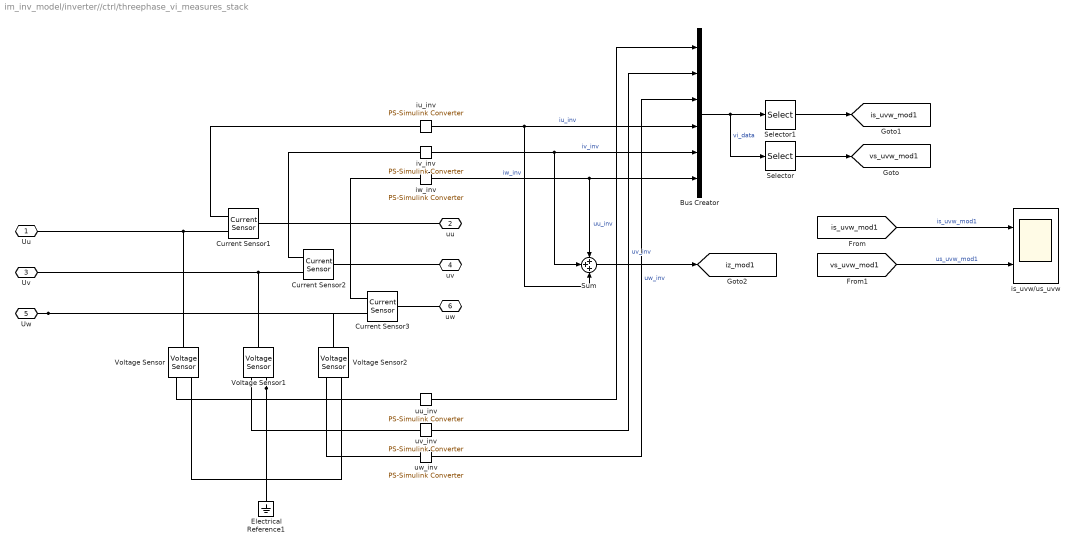
== system im_inv_model/inverter//ctrl/threephase_vi_measures_stack ==
  Bus Creator : BusCreator  Inputs=6
  Current Sensor1 : fl_lib/Electrical/Electrical Sensors/Current Sensor
  Current Sensor2 : fl_lib/Electrical/Electrical Sensors/Current Sensor
  Current Sensor3 : fl_lib/Electrical/Electrical Sensors/Current Sensor
  Electrical Reference1 : fl_lib/Electrical/Electrical Elements/Electrical Reference
  Selector : Selector  InputPortWidth=6  IndexOptions=Index vector (dialog)  Indices=[1 2 3]  OutputSizes=1
  Selector1 : Selector  InputPortWidth=6  IndexOptions=Index vector (dialog)  Indices=[4 5 6]  OutputSizes=1
  Sum : Sum  Inputs=+++
  Voltage Sensor : fl_lib/Electrical/Electrical Sensors/Voltage Sensor
  Voltage Sensor1 : fl_lib/Electrical/Electrical Sensors/Voltage Sensor
  Voltage Sensor2 : fl_lib/Electrical/Electrical Sensors/Voltage Sensor
  is_uvw/us_uvw : Scope  NumInputPorts=2
      settings: ActiveDisplayYMinimum=-947.9760634971849  ActiveDisplayYMaximum=948.24797756926182
  iu_inv : nesl_utility/PS-Simulink Converter  PhysicalDomain=network_engine_domain  SubClassName=ps_output  LeftPortType=input  RightPortType=output  PseudoPeriodic=off  Frequencies=[]  VectorFormat=1-D array  Unit=A  AffineConversion=off
  iv_inv : nesl_utility/PS-Simulink Converter  PhysicalDomain=network_engine_domain  SubClassName=ps_output  LeftPortType=input  RightPortType=output  PseudoPeriodic=off  Frequencies=[]  VectorFormat=1-D array  Unit=A  AffineConversion=off
  iw_inv : nesl_utility/PS-Simulink Converter  PhysicalDomain=network_engine_domain  SubClassName=ps_output  LeftPortType=input  RightPortType=output  PseudoPeriodic=off  Frequencies=[]  VectorFormat=1-D array  Unit=A  AffineConversion=off
  uu_inv : nesl_utility/PS-Simulink Converter  PhysicalDomain=network_engine_domain  SubClassName=ps_output  LeftPortType=input  RightPortType=output  PseudoPeriodic=off  Frequencies=[]  VectorFormat=1-D array  Unit=V  AffineConversion=off
  uv_inv : nesl_utility/PS-Simulink Converter  PhysicalDomain=network_engine_domain  SubClassName=ps_output  LeftPortType=input  RightPortType=output  PseudoPeriodic=off  Frequencies=[]  VectorFormat=1-D array  Unit=V  AffineConversion=off
  uw_inv : nesl_utility/PS-Simulink Converter  PhysicalDomain=network_engine_domain  SubClassName=ps_output  LeftPortType=input  RightPortType=output  PseudoPeriodic=off  Frequencies=[]  VectorFormat=1-D array  Unit=V  AffineConversion=off
  Uu : PMIOPort  Side=Left
  uu : PMIOPort  Port=2  Side=Right
  Uv : PMIOPort  Port=3  Side=Left
  uv : PMIOPort  Port=4  Side=Right
  Uw : PMIOPort  Port=5  Side=Left
  uw : PMIOPort  Port=6  Side=Right
  tag scope: is_uvw_mod1=global, iz_mod1=global, vs_uvw_mod1=global
  wires:
  [vs_uvw_mod1] -> is_uvw/us_uvw/2  "us_uvw_mod1"
  [is_uvw_mod1] -> is_uvw/us_uvw/1  "is_uvw_mod1"
  uw_inv/1 -> Bus Creator/3  "uw_inv"
  uv_inv/1 -> Bus Creator/2  "uv_inv"
  uu_inv/1 -> Bus Creator/1  "uu_inv"
  iw_inv/1 -> Sum/1, Bus Creator/6  "iw_inv"
  iu_inv/1 -> Bus Creator/4, Sum/3  "iu_inv"
  iv_inv/1 -> Bus Creator/5, Sum/2  "iv_inv"
  Selector/1 -> [vs_uvw_mod1]
  Bus Creator/1 -> Selector/1, Selector1/1  "vi_data"
  Selector1/1 -> [is_uvw_mod1]
  Sum/1 -> [iz_mod1]
  connections:
  uw/RConn1 -- Current Sensor3/LConn1
  Voltage Sensor2/RConn1 -- uw_inv/LConn1
  Voltage Sensor/LConn1 -- Current Sensor1/RConn2 -- Uu/RConn1
  Uw/RConn1 -- Current Sensor3/RConn2 -- Voltage Sensor2/LConn1
  Voltage Sensor1/RConn1 -- uv_inv/LConn1
  Voltage Sensor/RConn1 -- uu_inv/LConn1
  Voltage Sensor1/RConn2 -- Voltage Sensor2/RConn2 -- Voltage Sensor/RConn2 -- Electrical Reference1/LConn1
  Voltage Sensor1/LConn1 -- Current Sensor2/RConn2 -- Uv/RConn1
  Current Sensor2/LConn1 -- uv/RConn1
  Current Sensor1/LConn1 -- uu/RConn1
  Current Sensor1/RConn1 -- iu_inv/LConn1
  Current Sensor2/RConn1 -- iv_inv/LConn1
  Current Sensor3/RConn1 -- iw_inv/LConn1

== system im_inv_model/induction motor/control performance evaluation/adc2dq_s_1 ==
  abc : Inport
  Bus Creator : BusCreator  Inputs=2
  abc2alphabeta : MATLAB Function  TreatAsAtomicUnit=on  SystemSampleTime=param.glb_time.tc
  alphabeta2xieta : MATLAB Function  TreatAsAtomicUnit=on  SystemSampleTime=param.glb_time.tc
  dq : Outport
  tag scope: psi_s_alpha_im=global, psi_s_beta_im=global
  wires:
  abc2alphabeta/1(alpha) -> [psi_s_alpha_im], alphabeta2xieta/1(alpha)  "alpha"
  abc2alphabeta/2(beta) -> [psi_s_beta_im], alphabeta2xieta/2(beta)  "beta"
  abc/1 -> abc2alphabeta/1(abc)
  [theta_s_mod1] -> alphabeta2xieta/3(theta)
  alphabeta2xieta/1(d) -> Bus Creator/1  "d"
  alphabeta2xieta/2(q) -> Bus Creator/2  "q"
  Bus Creator/1 -> dq/1

== system im_inv_model/induction motor/control performance evaluation/adc2dq_s_2 ==
  abc : Inport
  Bus Creator : BusCreator  Inputs=2
  abc2alphabeta : MATLAB Function  TreatAsAtomicUnit=on  SystemSampleTime=param.glb_time.tc
  alphabeta2xieta : MATLAB Function  TreatAsAtomicUnit=on  SystemSampleTime=param.glb_time.tc
  dq : Outport
  wires:
  Bus Creator/1 -> dq/1
  alphabeta2xieta/2(q) -> Bus Creator/2  "q"
  alphabeta2xieta/1(d) -> Bus Creator/1  "d"
  [theta_s_mod1] -> alphabeta2xieta/3(theta)
  abc/1 -> abc2alphabeta/1(abc)
  abc2alphabeta/2(beta) -> alphabeta2xieta/2(beta)  "beta"
  abc2alphabeta/1(alpha) -> alphabeta2xieta/1(alpha)  "alpha"

== system im_inv_model/induction motor/control performance evaluation/adc2dq_slip_1 ==
  abc : Inport
  Bus Creator : BusCreator  Inputs=2
  abc2alphabeta : MATLAB Function  TreatAsAtomicUnit=on  SystemSampleTime=param.glb_time.tc
  alphabeta2xieta : MATLAB Function  TreatAsAtomicUnit=on  SystemSampleTime=param.glb_time.tc
  dq : Outport
  wires:
  Bus Creator/1 -> dq/1
  alphabeta2xieta/2(q) -> Bus Creator/2  "q"
  alphabeta2xieta/1(d) -> Bus Creator/1  "d"
  [theta_slip_mod1] -> alphabeta2xieta/3(theta)
  abc/1 -> abc2alphabeta/1(abc)
  abc2alphabeta/2(beta) -> alphabeta2xieta/2(beta)  "beta"
  abc2alphabeta/1(alpha) -> alphabeta2xieta/1(alpha)  "alpha"

== system im_inv_model/induction motor/control performance evaluation/adc2dq_slip_2 ==
  abc : Inport
  Bus Creator : BusCreator  Inputs=2
  abc2alphabeta : MATLAB Function  TreatAsAtomicUnit=on  SystemSampleTime=param.glb_time.tc
  alphabeta2xieta : MATLAB Function  TreatAsAtomicUnit=on  SystemSampleTime=param.glb_time.tc
  dq : Outport
  wires:
  abc2alphabeta/1(alpha) -> alphabeta2xieta/1(alpha)  "alpha"
  abc2alphabeta/2(beta) -> alphabeta2xieta/2(beta)  "beta"
  abc/1 -> abc2alphabeta/1(abc)
  [theta_slip_mod1] -> alphabeta2xieta/3(theta)
  alphabeta2xieta/1(d) -> Bus Creator/1  "d"
  alphabeta2xieta/2(q) -> Bus Creator/2  "q"
  Bus Creator/1 -> dq/1

== system im_inv_model/induction motor/mechanical data/double_integrator_observer_for_im ==
  theta : Inport
  Gain : Gain  Gain=param.im.ctrl.di_obs.Ldso  Multiplication=Matrix(K*u)
  Gain1 : Gain  Gain=param.im.ctrl.di_obs.Adso  Multiplication=Matrix(K*u)
  Gain2 : Gain  Gain=param.im.ctrl.di_obs.Cso  Multiplication=Matrix(K*u)
  Selector : Selector  InputPortWidth=2  IndexOptions=Index vector (dialog)  Indices=2  OutputSizes=1
  Sum : Sum  Inputs=-+|
  Sum1 : Sum  Inputs=|++
  Unit Delay : UnitDelay  SampleTime=param.glb_time.ts_inv
  bounder1 : MATLAB Function  TreatAsAtomicUnit=on  SystemSampleTime=param.glb_time.ts_inv
  bounder2 : MATLAB Function  TreatAsAtomicUnit=on  SystemSampleTime=param.glb_time.ts_inv
  omega_hat : Outport
  wires:
  Gain/1 -> Sum1/1
  Selector/1 -> omega_hat/1
  Gain2/1 -> bounder2/1(u)  "theta_hat"
  Gain1/1 -> Sum1/2
  Sum1/1 -> Unit Delay/1
  Sum/1 -> bounder1/1(u)
  Unit Delay/1 -> Gain1/1, Selector/1, Gain2/1
  theta/1 -> Sum/2  "theta"
  bounder1/1(y) -> Gain/1
  bounder2/1(y) -> Sum/1  "theta_hat_bounded"

== system im_inv_model/induction motor/mechanical data/encoder_measure ==
  Gain1 : Gain  Gain=param.im.machine.pp
  Zero-Order Hold1 : ZeroOrderHold  SampleTime=param.glb_time.ts_inv
  bounder2 : MATLAB Function  TreatAsAtomicUnit=on  SystemSampleTime=param.glb_time.ts_inv
  rotor_phase_elec_encoder : Outport
  wires:
  bounder2/1(y) -> rotor_phase_elec_encoder/1
  Zero-Order Hold1/1 -> Gain1/1
  Gain1/1 -> bounder2/1(u)
  [rotor_phase_m_encoder] -> Zero-Order Hold1/1

== system im_inv_model/inverter//ctrl/im_ctrl/abc2dq ==
  a : Inport
  b : Inport  Port=2
  c : Inport  Port=3
  wt : Inport  Port=4
  To Workspace1 : ToWorkspace  VariableName=is_beta_mod1_sim  SampleTime=param.glb_time.tc
      settings: MaxDataPoints=param.glb_time.Nc  Decimation=param.glb_time.decimation_tc
  To Workspace2 : ToWorkspace  VariableName=is_alpha_mod1_sim  SampleTime=param.glb_time.tc
      settings: MaxDataPoints=param.glb_time.Nc  Decimation=param.glb_time.decimation_tc
  abc2alphabeta : Subsystem
  alphabeta2dq : Subsystem
  d : Outport  VectorParamsAs1DForOutWhenUnconnected=off
  q : Outport  Port=2  VectorParamsAs1DForOutWhenUnconnected=off
  tag scope: is_alpha_pu_mod1=global, is_beta_pu_mod1=global
  wires:
  wt/1 -> alphabeta2dq/3(wt)
  b/1 -> abc2alphabeta/2(b)
  c/1 -> abc2alphabeta/3(c)
  a/1 -> abc2alphabeta/1(a)
  alphabeta2dq/1(d) -> d/1
  alphabeta2dq/2(q) -> q/1
  abc2alphabeta/1("alpha ") -> [is_alpha_pu_mod1], alphabeta2dq/1(alpha), To Workspace2/1
  abc2alphabeta/2("beta ") -> [is_beta_pu_mod1], alphabeta2dq/2(beta), To Workspace1/1
